simulink model "Euler"  (R2023b)
settings: Solver=VariableStepAuto  StartTime=0.0  StopTime=150  RelTol=1e-3
values from neighbouring files (symbols this model uses):
  c2_init = c2_0    (= 4)    [tank_model.m]
  c3_init = c3_0    (= 4.2)    [tank_model.m]
  h1_init = h1_0    (= 0.75)    [tank_model.m]
  h2_init = h2_0    (= 0.7)    [tank_model.m]
  h3_init = h3_0    (= 0.85)    [tank_model.m]
  sample_time = 0.5    [tank_model.m]
undefined symbols (not defined in the file or in its folder): DiscIntNeverNeededParam, params
libraries: slpidlib x4
settings Model: Creator=fyder9  LastModifiedBy=fyder9

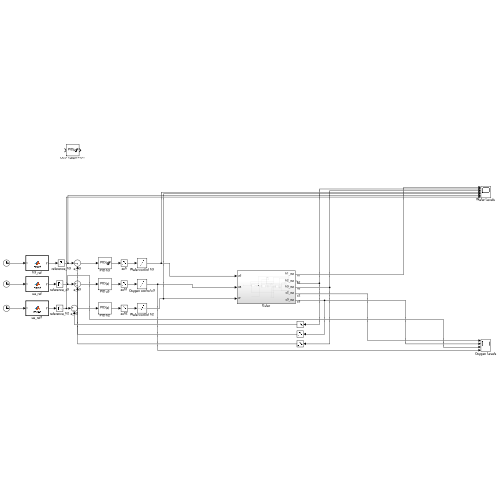
[thumbnail: Simulink's stored preview of the top-level diagram]
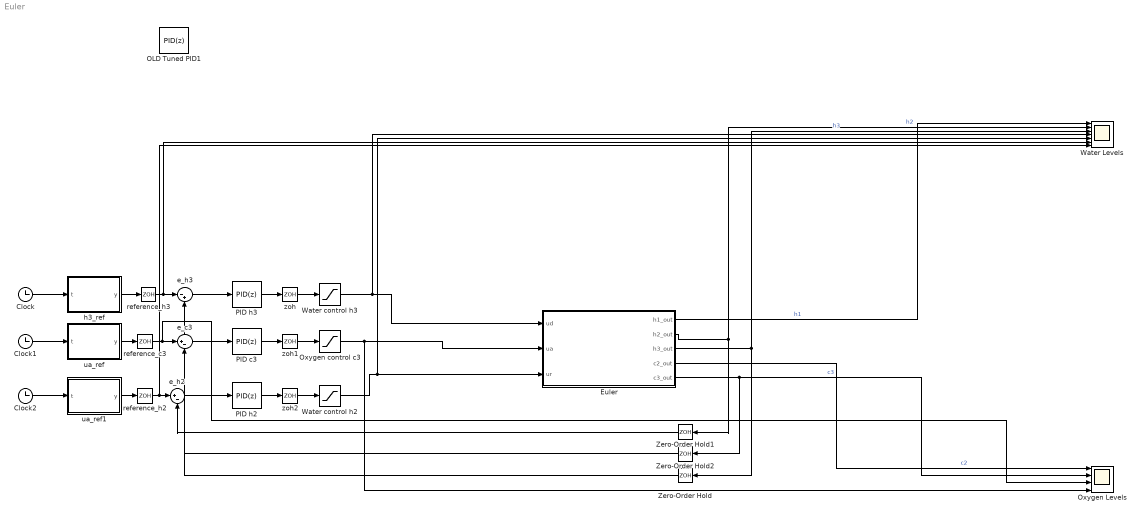
== system Euler ==
  Clock : Clock
  Clock1 : Clock
  Clock2 : Clock
  Euler : Subsystem
  OLD Tuned PID1 : slpidlib/PID Controller  Controller=PID  Form=Parallel  TimeDomain=Discrete-time  UseExternalTs=off  SampleTime=-1  IntegratorMethod=Forward Euler  FilterMethod=Forward Euler  ControllerParametersSource=internal  P=4.67716748427759  I=1.09175963093947  UseKiTs=off  D=3.88894553033778  N=6.50572443588666  UseFilter=on  TunerSelectOption=Transfer Function Based (PID Tuner App)  InitialConditionSource=internal  InitialConditionForIntegrator=0  InitialConditionForFilter=0  DifferentiatorICPrevScaledInput=0  ExternalReset=none  TrackingMode=off  Kt=1  LimitOutput=on  SatLimitsSource=internal  UpperSaturationLimit=inf  LowerSaturationLimit=-inf  LinearizeAsGain=on  AntiWindupMode=clamping  Kb=1  LimitIntegrator=off  UpperIntegratorSaturationLimit=inf  LowerIntegratorSaturationLimit=-inf  POutMin=[]  POutMax=[]  IOutMin=[]  IOutMax=[]  DOutMin=[]  DOutMax=[]  NOutMin=[]  NOutMax=[]  SumOutMin=[]  SumOutMax=[]  SaturationOutMin=[]  SaturationOutMax=[]  PParamMin=[]  PParamMax=[]  IParamMin=[]  IParamMax=[]  DParamMin=[]  DParamMax=[]  NParamMin=[]  NParamMax=[]  KbParamMin=[]  KbParamMax=[]  KtParamMin=[]  KtParamMax=[]  KbOutMin=[]  KbOutMax=[]  KtOutMin=[]  KtOutMax=[]  IntegratorOutMin=[]  IntegratorOutMax=[]  FilterOutMin=[]  FilterOutMax=[]  SumI1OutMin=[]  SumI1OutMax=[]  SumI2OutMin=[]  SumI2OutMax=[]  SumI3OutMin=[]  SumI3OutMax=[]  SumI4OutMin=[]  SumI4OutMax=[]  SumDOutMin=[]  SumDOutMax=[]  DifferentiatorOutMin=[]  DifferentiatorOutMax=[]  FilterDiffOutCoefMin=[]  FilterDiffOutCoefMax=[]  ReciprocalOutMin=[]  ReciprocalOutMax=[]  SumDenOutMin=[]  SumDenOutMax=[]  SumNumOutMin=[]  SumNumOutMax=[]  DivideOutMin=[]  DivideOutMax=[]  UdiffTsProdOutMin=[]  UdiffTsProdOutMax=[]  NTsProdOutMin=[]  NTsProdOutMax=[]  UintegralTsProdOutMin=[]  UintegralTsProdOutMax=[]  UngainTsProdOutMin=[]  UngainTsProdOutMax=[]  ClampingZeroOutDataTypeStr=Inherit: Inherit via back propagation  ClampingZeroOutMin=[]  ClampingZeroOutMax=[]  FilterDenConstantOutDataTypeStr=Inherit: Inherit via back propagation  FilterDenConstantOutMin=[]  FilterDenConstantOutMax=[]  PCopyOutDataTypeStr=Inherit: Inherit via back propagation  PCopyOutMin=[]  PCopyOutMax=[]  NCopyOutDataTypeStr=Inherit: Inherit via back propagation  NCopyOutMin=[]  NCopyOutMax=[]  IntegratorContinuousStateAttributes=''  IntegratorStateMustResolveToSignalObject=off  IntegratorRTWStateStorageClass=Auto  FilterContinuousStateAttributes=''  FilterStateMustResolveToSignalObject=off  FilterRTWStateStorageClass=Auto  ParallelPVariant=InternalParameters  IdealPVariant=Disabled  IVariant=InternalParameters  DVariant=InternalParameters  IntegratorVariant=Discrete  SatVariant=Enabled  AWVariant=DiscClampingParallel  PCopyVariant=Disabled  TRVariant=Disabled  FdbkBlocksVariant=Forward  IdealPFdbkVariant=Disabled  SatFdbkVariant=Disabled  DerivativeFilterVariant=ForwardEulerFilter  NVariant=InternalParameters  NCopyVariant=Disabled  FilterICVariant=InternalICsFilter  IntegratorICVariant=InternalICs  ExternalResetVariant=Disabled  TRSumVariant=Passthrough  SumFdbkVariant=Disabled  SumVariant=Sum_PID  TsampFilterVariant=InternalTs  TsampNgainVariant=Passthrough  TsampIntegralVariant=Disabled_SignalSpec  ExternalSaturationOutDataTypeStr=Inherit: Same as second input
  Oxygen Levels : Scope  NumInputPorts=4
  Oxygen control c3 : Saturate  UpperLimit=1  LowerLimit=0  LinearizeAsGain=off
  PID c3 : slpidlib/PID Controller  Controller=PID  Form=Parallel  TimeDomain=Discrete-time  UseExternalTs=off  SampleTime=-1  IntegratorMethod=Forward Euler  FilterMethod=Forward Euler  ControllerParametersSource=internal  P=0.1  I=0.02  UseKiTs=off  D=0  N=100  UseFilter=on  TunerSelectOption=Transfer Function Based (PID Tuner App)  InitialConditionSource=internal  InitialConditionForIntegrator=0  InitialConditionForFilter=0  DifferentiatorICPrevScaledInput=0  ExternalReset=none  TrackingMode=off  Kt=1  LimitOutput=off  SatLimitsSource=internal  UpperSaturationLimit=inf  LowerSaturationLimit=-inf  LinearizeAsGain=off  AntiWindupMode=none  Kb=1  LimitIntegrator=off  UpperIntegratorSaturationLimit=inf  LowerIntegratorSaturationLimit=-inf  POutMin=[]  POutMax=[]  IOutMin=[]  IOutMax=[]  DOutMin=[]  DOutMax=[]  NOutMin=[]  NOutMax=[]  SumOutMin=[]  SumOutMax=[]  SaturationOutMin=[]  SaturationOutMax=[]  PParamMin=[]  PParamMax=[]  IParamMin=[]  IParamMax=[]  DParamMin=[]  DParamMax=[]  NParamMin=[]  NParamMax=[]  KbParamMin=[]  KbParamMax=[]  KtParamMin=[]  KtParamMax=[]  KbOutMin=[]  KbOutMax=[]  KtOutMin=[]  KtOutMax=[]  IntegratorOutMin=[]  IntegratorOutMax=[]  FilterOutMin=[]  FilterOutMax=[]  SumI1OutMin=[]  SumI1OutMax=[]  SumI2OutMin=[]  SumI2OutMax=[]  SumI3OutMin=[]  SumI3OutMax=[]  SumI4OutMin=[]  SumI4OutMax=[]  SumDOutMin=[]  SumDOutMax=[]  DifferentiatorOutMin=[]  DifferentiatorOutMax=[]  FilterDiffOutCoefMin=[]  FilterDiffOutCoefMax=[]  ReciprocalOutMin=[]  ReciprocalOutMax=[]  SumDenOutMin=[]  SumDenOutMax=[]  SumNumOutMin=[]  SumNumOutMax=[]  DivideOutMin=[]  DivideOutMax=[]  UdiffTsProdOutMin=[]  UdiffTsProdOutMax=[]  NTsProdOutMin=[]  NTsProdOutMax=[]  UintegralTsProdOutMin=[]  UintegralTsProdOutMax=[]  UngainTsProdOutMin=[]  UngainTsProdOutMax=[]  ClampingZeroOutDataTypeStr=Inherit: Inherit via back propagation  ClampingZeroOutMin=[]  ClampingZeroOutMax=[]  FilterDenConstantOutDataTypeStr=Inherit: Inherit via back propagation  FilterDenConstantOutMin=[]  FilterDenConstantOutMax=[]  PCopyOutDataTypeStr=Inherit: Inherit via back propagation  PCopyOutMin=[]  PCopyOutMax=[]  NCopyOutDataTypeStr=Inherit: Inherit via back propagation  NCopyOutMin=[]  NCopyOutMax=[]  IntegratorContinuousStateAttributes=''  IntegratorStateMustResolveToSignalObject=off  IntegratorRTWStateStorageClass=Auto  FilterContinuousStateAttributes=''  FilterStateMustResolveToSignalObject=off  FilterRTWStateStorageClass=Auto  ParallelPVariant=InternalParameters  IdealPVariant=Disabled  IVariant=InternalParameters  DVariant=InternalParameters  IntegratorVariant=Discrete  SatVariant=Disabled  AWVariant=Passthrough  PCopyVariant=Disabled  TRVariant=Disabled  FdbkBlocksVariant=Forward  IdealPFdbkVariant=Disabled  SatFdbkVariant=Disabled  DerivativeFilterVariant=ForwardEulerFilter  NVariant=InternalParameters  NCopyVariant=Disabled  FilterICVariant=InternalICsFilter  IntegratorICVariant=InternalICs  ExternalResetVariant=Disabled  TRSumVariant=Passthrough  SumFdbkVariant=Disabled  SumVariant=Sum_PID  TsampFilterVariant=InternalTs  TsampNgainVariant=Passthrough  TsampIntegralVariant=Disabled_SignalSpec  ExternalSaturationOutDataTypeStr=Inherit: Same as second input
      settings: LibrarySourceBlock=simulink/Discrete/Discrete PID Controller
  PID h2 : slpidlib/PID Controller  Controller=PID  Form=Parallel  TimeDomain=Discrete-time  UseExternalTs=off  SampleTime=-1  IntegratorMethod=Forward Euler  FilterMethod=Forward Euler  ControllerParametersSource=internal  P=0.2  I=0.03  UseKiTs=off  D=0  N=100  UseFilter=on  TunerSelectOption=Transfer Function Based (PID Tuner App)  InitialConditionSource=internal  InitialConditionForIntegrator=0  InitialConditionForFilter=0  DifferentiatorICPrevScaledInput=0  ExternalReset=none  TrackingMode=off  Kt=1  LimitOutput=off  SatLimitsSource=internal  UpperSaturationLimit=inf  LowerSaturationLimit=-inf  LinearizeAsGain=off  AntiWindupMode=none  Kb=1  LimitIntegrator=off  UpperIntegratorSaturationLimit=inf  LowerIntegratorSaturationLimit=-inf  POutMin=[]  POutMax=[]  IOutMin=[]  IOutMax=[]  DOutMin=[]  DOutMax=[]  NOutMin=[]  NOutMax=[]  SumOutMin=[]  SumOutMax=[]  SaturationOutMin=[]  SaturationOutMax=[]  PParamMin=[]  PParamMax=[]  IParamMin=[]  IParamMax=[]  DParamMin=[]  DParamMax=[]  NParamMin=[]  NParamMax=[]  KbParamMin=[]  KbParamMax=[]  KtParamMin=[]  KtParamMax=[]  KbOutMin=[]  KbOutMax=[]  KtOutMin=[]  KtOutMax=[]  IntegratorOutMin=[]  IntegratorOutMax=[]  FilterOutMin=[]  FilterOutMax=[]  SumI1OutMin=[]  SumI1OutMax=[]  SumI2OutMin=[]  SumI2OutMax=[]  SumI3OutMin=[]  SumI3OutMax=[]  SumI4OutMin=[]  SumI4OutMax=[]  SumDOutMin=[]  SumDOutMax=[]  DifferentiatorOutMin=[]  DifferentiatorOutMax=[]  FilterDiffOutCoefMin=[]  FilterDiffOutCoefMax=[]  ReciprocalOutMin=[]  ReciprocalOutMax=[]  SumDenOutMin=[]  SumDenOutMax=[]  SumNumOutMin=[]  SumNumOutMax=[]  DivideOutMin=[]  DivideOutMax=[]  UdiffTsProdOutMin=[]  UdiffTsProdOutMax=[]  NTsProdOutMin=[]  NTsProdOutMax=[]  UintegralTsProdOutMin=[]  UintegralTsProdOutMax=[]  UngainTsProdOutMin=[]  UngainTsProdOutMax=[]  ClampingZeroOutDataTypeStr=Inherit: Inherit via back propagation  ClampingZeroOutMin=[]  ClampingZeroOutMax=[]  FilterDenConstantOutDataTypeStr=Inherit: Inherit via back propagation  FilterDenConstantOutMin=[]  FilterDenConstantOutMax=[]  PCopyOutDataTypeStr=Inherit: Inherit via back propagation  PCopyOutMin=[]  PCopyOutMax=[]  NCopyOutDataTypeStr=Inherit: Inherit via back propagation  NCopyOutMin=[]  NCopyOutMax=[]  IntegratorContinuousStateAttributes=''  IntegratorStateMustResolveToSignalObject=off  IntegratorRTWStateStorageClass=Auto  FilterContinuousStateAttributes=''  FilterStateMustResolveToSignalObject=off  FilterRTWStateStorageClass=Auto  ParallelPVariant=InternalParameters  IdealPVariant=Disabled  IVariant=InternalParameters  DVariant=InternalParameters  IntegratorVariant=Discrete  SatVariant=Disabled  AWVariant=Passthrough  PCopyVariant=Disabled  TRVariant=Disabled  FdbkBlocksVariant=Forward  IdealPFdbkVariant=Disabled  SatFdbkVariant=Disabled  DerivativeFilterVariant=ForwardEulerFilter  NVariant=InternalParameters  NCopyVariant=Disabled  FilterICVariant=InternalICsFilter  IntegratorICVariant=InternalICs  ExternalResetVariant=Disabled  TRSumVariant=Passthrough  SumFdbkVariant=Disabled  SumVariant=Sum_PID  TsampFilterVariant=InternalTs  TsampNgainVariant=Passthrough  TsampIntegralVariant=Disabled_SignalSpec  ExternalSaturationOutDataTypeStr=Inherit: Same as second input
      settings: LibrarySourceBlock=simulink/Discrete/Discrete PID Controller
  PID h3 : slpidlib/PID Controller  Controller=PID  Form=Parallel  TimeDomain=Discrete-time  UseExternalTs=off  SampleTime=-1  IntegratorMethod=Forward Euler  FilterMethod=Forward Euler  ControllerParametersSource=internal  P=0.6  I=0.08  UseKiTs=off  D=0  N=100  UseFilter=on  TunerSelectOption=Transfer Function Based (PID Tuner App)  InitialConditionSource=internal  InitialConditionForIntegrator=0  InitialConditionForFilter=0  DifferentiatorICPrevScaledInput=0  ExternalReset=none  TrackingMode=off  Kt=1  LimitOutput=on  SatLimitsSource=internal  UpperSaturationLimit=inf  LowerSaturationLimit=-inf  LinearizeAsGain=off  AntiWindupMode=clamping  Kb=1  LimitIntegrator=off  UpperIntegratorSaturationLimit=inf  LowerIntegratorSaturationLimit=-inf  POutMin=[]  POutMax=[]  IOutMin=[]  IOutMax=[]  DOutMin=[]  DOutMax=[]  NOutMin=[]  NOutMax=[]  SumOutMin=[]  SumOutMax=[]  SaturationOutMin=[]  SaturationOutMax=[]  PParamMin=[]  PParamMax=[]  IParamMin=[]  IParamMax=[]  DParamMin=[]  DParamMax=[]  NParamMin=[]  NParamMax=[]  KbParamMin=[]  KbParamMax=[]  KtParamMin=[]  KtParamMax=[]  KbOutMin=[]  KbOutMax=[]  KtOutMin=[]  KtOutMax=[]  IntegratorOutMin=[]  IntegratorOutMax=[]  FilterOutMin=[]  FilterOutMax=[]  SumI1OutMin=[]  SumI1OutMax=[]  SumI2OutMin=[]  SumI2OutMax=[]  SumI3OutMin=[]  SumI3OutMax=[]  SumI4OutMin=[]  SumI4OutMax=[]  SumDOutMin=[]  SumDOutMax=[]  DifferentiatorOutMin=[]  DifferentiatorOutMax=[]  FilterDiffOutCoefMin=[]  FilterDiffOutCoefMax=[]  ReciprocalOutMin=[]  ReciprocalOutMax=[]  SumDenOutMin=[]  SumDenOutMax=[]  SumNumOutMin=[]  SumNumOutMax=[]  DivideOutMin=[]  DivideOutMax=[]  UdiffTsProdOutMin=[]  UdiffTsProdOutMax=[]  NTsProdOutMin=[]  NTsProdOutMax=[]  UintegralTsProdOutMin=[]  UintegralTsProdOutMax=[]  UngainTsProdOutMin=[]  UngainTsProdOutMax=[]  ClampingZeroOutDataTypeStr=Inherit: Inherit via back propagation  ClampingZeroOutMin=[]  ClampingZeroOutMax=[]  FilterDenConstantOutDataTypeStr=Inherit: Inherit via back propagation  FilterDenConstantOutMin=[]  FilterDenConstantOutMax=[]  PCopyOutDataTypeStr=Inherit: Inherit via back propagation  PCopyOutMin=[]  PCopyOutMax=[]  NCopyOutDataTypeStr=Inherit: Inherit via back propagation  NCopyOutMin=[]  NCopyOutMax=[]  IntegratorContinuousStateAttributes=''  IntegratorStateMustResolveToSignalObject=off  IntegratorRTWStateStorageClass=Auto  FilterContinuousStateAttributes=''  FilterStateMustResolveToSignalObject=off  FilterRTWStateStorageClass=Auto  ParallelPVariant=InternalParameters  IdealPVariant=Disabled  IVariant=InternalParameters  DVariant=InternalParameters  IntegratorVariant=Discrete  SatVariant=Enabled  AWVariant=DiscClampingParallel  PCopyVariant=Disabled  TRVariant=Disabled  FdbkBlocksVariant=Forward  IdealPFdbkVariant=Disabled  SatFdbkVariant=Disabled  DerivativeFilterVariant=ForwardEulerFilter  NVariant=InternalParameters  NCopyVariant=Disabled  FilterICVariant=InternalICsFilter  IntegratorICVariant=InternalICs  ExternalResetVariant=Disabled  TRSumVariant=Passthrough  SumFdbkVariant=Disabled  SumVariant=Sum_PID  TsampFilterVariant=InternalTs  TsampNgainVariant=Passthrough  TsampIntegralVariant=Disabled_SignalSpec  ExternalSaturationOutDataTypeStr=Inherit: Same as second input
      settings: LibrarySourceBlock=simulink/Discrete/Discrete PID Controller
  Water Levels : Scope  NumInputPorts=7
  Water control h2 : Saturate  UpperLimit=0.25  LowerLimit=0.05  LinearizeAsGain=off
  Water control h3 : Saturate  UpperLimit=0.25  LowerLimit=0.05  LinearizeAsGain=off
  Zero-Order Hold : ZeroOrderHold  SampleTime=0.5
  Zero-Order Hold1 : ZeroOrderHold  SampleTime=0.5
  Zero-Order Hold2 : ZeroOrderHold  SampleTime=0.5
  e_c3 : Sum  Inputs=|+-
  e_h2 : Sum  Inputs=|+-
  e_h3 : Sum  Inputs=|-+
  h3_ref : MATLAB Function  TreatAsAtomicUnit=on
  reference_c3 : ZeroOrderHold  SampleTime=0.5
  reference_h2 : ZeroOrderHold  SampleTime=0.5
  reference_h3 : ZeroOrderHold  SampleTime=0.5
  ua_ref : MATLAB Function  TreatAsAtomicUnit=on
  ua_ref1 : MATLAB Function  TreatAsAtomicUnit=on
  zoh : ZeroOrderHold  SampleTime=0.5
  zoh1 : ZeroOrderHold  SampleTime=0.5
  zoh2 : ZeroOrderHold  SampleTime=0.5
  wires:
  e_h2/1 -> PID h2/1
  Euler/2(h2_out) -> Water Levels/2, Zero-Order Hold1/1  "h2"
  Euler/3(h3_out) -> Water Levels/3, Zero-Order Hold/1  "h3"
  Euler/4(c2_out) -> Oxygen Levels/1  "c2"
  Euler/5(c3_out) -> Zero-Order Hold2/1, Oxygen Levels/2  "c3"
  h3_ref/1(y) -> reference_h3/1
  e_h3/1 -> PID h3/1
  ua_ref/1(y) -> reference_c3/1
  e_c3/1 -> PID c3/1
  Clock/1 -> h3_ref/1(t)
  Clock1/1 -> ua_ref/1(t)
  Water control h3/1 -> Euler/1(ud), Water Levels/4
  PID c3/1 -> zoh1/1
  Oxygen control c3/1 -> Oxygen Levels/4, Euler/2(ua)
  PID h3/1 -> zoh/1
  Clock2/1 -> ua_ref1/1(t)
  ua_ref1/1(y) -> reference_h2/1
  PID h2/1 -> zoh2/1
  Water control h2/1 -> Euler/3(ur), Water Levels/5
  Euler/1(h1_out) -> Water Levels/1  "h1"
  Zero-Order Hold1/1 -> e_h2/2
  Zero-Order Hold/1 -> e_h3/2
  Zero-Order Hold2/1 -> e_c3/2
  reference_h2/1 -> Water Levels/7, e_h2/1
  reference_c3/1 -> Oxygen Levels/3, e_c3/1
  reference_h3/1 -> Water Levels/6, e_h3/1
  zoh/1 -> Water control h3/1
  zoh1/1 -> Oxygen control c3/1
  zoh2/1 -> Water control h2/1

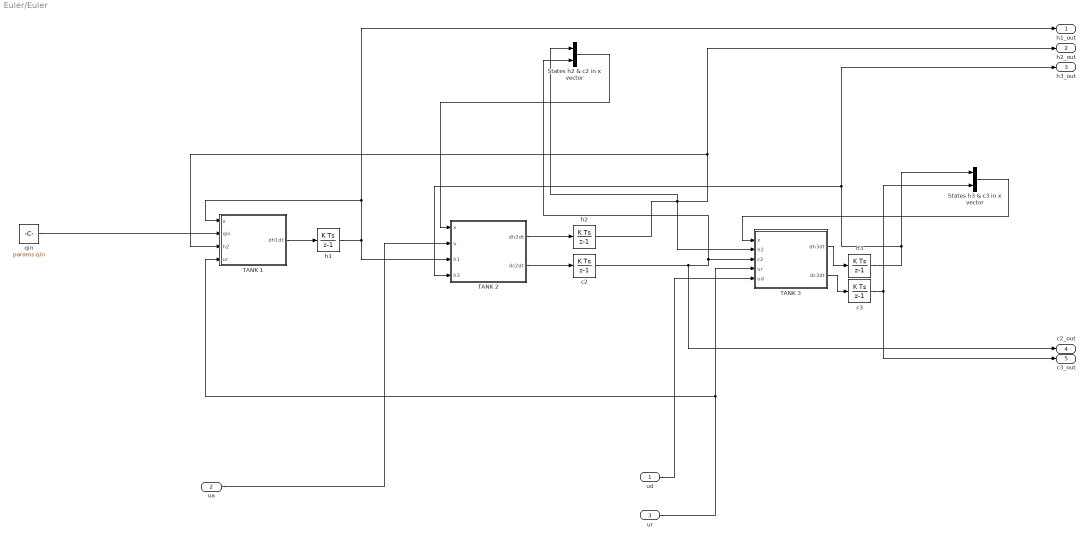
== system Euler/Euler ==
  ud : Inport
  ua : Inport  Port=2
  ur : Inport  Port=3
  States h2 & c2 in x vector : Mux  Inputs=2
  States h3 & c3 in x vector : Mux  Inputs=2
  TANK 1 : MATLAB Function  TreatAsAtomicUnit=on
  TANK 2 : MATLAB Function  TreatAsAtomicUnit=on
  TANK 3 : MATLAB Function  TreatAsAtomicUnit=on
  c2 : DiscreteIntegrator  InitialCondition=c2_init  SampleTime=sample_time  LimitOutput=on  LowerSaturationLimit=0  ICPrevOutput=DiscIntNeverNeededParam  ICPrevScaledInput=DiscIntNeverNeededParam
  c3 : DiscreteIntegrator  InitialCondition=c3_init  SampleTime=sample_time  LimitOutput=on  LowerSaturationLimit=0  ICPrevOutput=DiscIntNeverNeededParam  ICPrevScaledInput=DiscIntNeverNeededParam
  h1 : DiscreteIntegrator  InitialCondition=h1_init  SampleTime=sample_time  LimitOutput=on  LowerSaturationLimit=0  ICPrevOutput=DiscIntNeverNeededParam  ICPrevScaledInput=DiscIntNeverNeededParam
  h2 : DiscreteIntegrator  InitialCondition=h2_init  SampleTime=sample_time  LimitOutput=on  LowerSaturationLimit=0  ICPrevOutput=DiscIntNeverNeededParam  ICPrevScaledInput=DiscIntNeverNeededParam
  h3 : DiscreteIntegrator  InitialCondition=h3_init  SampleTime=sample_time  LimitOutput=on  LowerSaturationLimit=0  ICPrevOutput=DiscIntNeverNeededParam  ICPrevScaledInput=DiscIntNeverNeededParam
  qin : Constant  Value=params.qin
  h1_out : Outport
  h2_out : Outport  Port=2
  h3_out : Outport  Port=3
  c2_out : Outport  Port=4
  c3_out : Outport  Port=5
  wires:
  ua/1 -> TANK 2/2(u)
  ur/1 -> TANK 1/4(ur), TANK 3/4(ur)
  States h2 & c2 in x vector/1 -> TANK 2/1(x)
  TANK 2/2(dc2dt) -> c2/1
  c2/1 -> c2_out/1, States h2 & c2 in x vector/2, TANK 3/3(c2)
  c3/1 -> c3_out/1, States h3 & c3 in x vector/2
  TANK 2/1(dh2dt) -> h2/1
  TANK 1/1(dh1dt) -> h1/1
  TANK 3/1(dh3dt) -> h3/1
  TANK 3/2(dc3dt) -> c3/1
  h3/1 -> h3_out/1, TANK 2/4(h3), States h3 & c3 in x vector/1
  h2/1 -> h2_out/1, TANK 1/3(h2), TANK 3/2(h2), States h2 & c2 in x vector/1
  States h3 & c3 in x vector/1 -> TANK 3/1(x)
  qin/1 -> TANK 1/2(qin)
  h1/1 -> TANK 2/3(h1), h1_out/1, TANK 1/1(x)
  ud/1 -> TANK 3/5(ud)

== matlab function Euler/ua_ref ==
  data: t input; y output
function y = c3ref(t)

y = 5.50 + 0.70*(1 - exp(-t/40)) + 0.20*sin(2*pi/75 * t);

== matlab function Euler/h3_ref ==
  data: t input; y output
function y = h3ref(t)

y = 0.90 + 0.06*sin(2*pi/90 * t + pi/4);

== matlab function Euler/ua_ref1 ==
  data: t input; y output
function y = h2ref(t)

y = 0.80 + 0.08*sin((2*pi/60)*t);

== matlab function Euler/TANK 1 ==
  data: x input; qin input; dh1dt output size=1; h2 input; ur input
function dh1dt = tank1(x, qin, h2, ur)
%state
%h1 = max(x, 1e-3);
h1 = x;
%params
A1 = 1.2;
k12 = 0.22;
%input ur
%flow rate
q12 = k12 * sqrt(max(h1 - h2, 0));
%q12 = min(q12, h1*A1);
dh1dt = (1/A1) * (qin + ur - q12);
end

== matlab function Euler/TANK 2 ==
  data: x input; u input; dh2dt output size=1; h1 input; h3 input; dc2dt output size=1
function [dh2dt, dc2dt] = tank2(x, u, h1, h3)

%states
h2 = max(x(1), 1e-3);
c2 = max(x(2), 0);
%params
A1 = 1.2;
A2 = 1.0;
cin = 1.0;
k12 = 0.22;
k23 = 0.20;
csat = 8.0;
lambda2 = 0.08;
ka = 0.9;
%input
ua = u;
%flow
q12 = k12 * sqrt(max(h1 - h2, 0));
q23 = k23 * sqrt(max(h2 - h3, 0));
%q23 = min(q23, h2*A2);
eps_h = 1e-2;
%output
dh2dt = (1/A2) * (q12 - q23);
dc2dt = (q12 / (A2 * max(h2, eps_h))) * (cin - c2) + ka * ua * (csat - c2) - lambda2 * c2;
end

== matlab function Euler/TANK 3 ==
  data: x input; dh3dt output size=1; h2 input; c2 input; dc3dt output size=1; ur input; ud input
function [dh3dt, dc3dt] = tank3(x, h2, c2, ur , ud)

%states
c3 = x(2);
h3 = max(x(1),1e-3);
%params
A2 = 1.0;
A3 = 1.4;
lambda3 = 0.05;
k23 = 0.20;
%flow
q23 = k23 * sqrt(max(h2 - h3, 0));
%q23 = min(q23, h2*A2);
eps_h = 1e-4;
%output
dh3dt = (1/A3) * (q23 - ud - ur);
dc3dt = (q23 / (A3 * max(h3, eps_h))) * (c2 - c3) - lambda3 * c3;

end
